simulink model "generic_src"  (Simulink 10.3)
settings: Solver=ode45  StartTime=0.0  StopTime=inf  RelTol=1e-3  EnableMultiTasking=on
undefined symbols (not defined in the file or in its folder): Area_Front, Area_Rear, ay_max_off, ay_max_on, ay_per_mu_max_off, ay_per_mu_max_on, Brake_ratio, brake_valve_ctrl_kP, cat1mode1_higher, cat1mode1_lower, cat1mode2_higher, cat1mode2_lower, cat1mode3_higher, cat1mode3_lower, cat2mode1_higher, cat2mode1_lower, cat2mode2_higher, cat2mode2_lower, cat2mode3_higher, cat2mode3_lower, delta_vel, diff_lock_fac, diff_lock_off, diff_lock_on, ESP_ctrl_kD, ESP_ctrl_kI, ESP_ctrl_kP, ESP_ctrl_restore_kI, ESP_min_throttle_fac, f_ax, f_slip, g, higherlimit_highvel, higherlimit_lowvel, highervel_fac, highervelocity_fac, InitialConditionForIntegrator, limit_acc, limit_selectlow, limit_starting, limit_vdiff, locktime_throttle, lowerlimit_highvel, lowerlimit_lowvel, lowervel_fac, lowervelocity_fac, min_throttle, MPS2KMPH, MSR_ctrl_kD, MSR_ctrl_kI, MSR_ctrl_kP, MSR_min_throttle_fac, PID_kP_sideslip, PID_kP_yawrate, RADpS2RpM, rBrake, RpM2RADpS, SH_SL_switch, sideslip_vel_corr, sidesplip_deviation_max ... (+35)
libraries: CarMaker4SL x136, simulink x55, simulink_extras x6
(part 6 of 9)

== system generic_src/CarMaker/IPG Vehicle/PowerTrain/PTControl Example/PTControl_In/CreateBus PTC_Cfg Gearbox10 ==
  In : Inport
  BusCreator : BusCreator  Inputs=38
  Demux : Demux  Outputs=38
      settings: DisplayOption=none
  Out : Outport  VectorParamsAs1DForOutWhenUnconnected=off
  wires:
  Demux/38 -> BusCreator/38  "PTC_Cfg Gearbox10 iBGear16"
  Demux/37 -> BusCreator/37  "PTC_Cfg Gearbox10 iBGear15"
  Demux/36 -> BusCreator/36  "PTC_Cfg Gearbox10 iBGear14"
  Demux/35 -> BusCreator/35  "PTC_Cfg Gearbox10 iBGear13"
  Demux/34 -> BusCreator/34  "PTC_Cfg Gearbox10 iBGear12"
  Demux/33 -> BusCreator/33  "PTC_Cfg Gearbox10 iBGear11"
  Demux/32 -> BusCreator/32  "PTC_Cfg Gearbox10 iBGear10"
  Demux/31 -> BusCreator/31  "PTC_Cfg Gearbox10 iBGear9"
  Demux/30 -> BusCreator/30  "PTC_Cfg Gearbox10 iBGear8"
  Demux/29 -> BusCreator/29  "PTC_Cfg Gearbox10 iBGear7"
  Demux/28 -> BusCreator/28  "PTC_Cfg Gearbox10 iBGear6"
  Demux/27 -> BusCreator/27  "PTC_Cfg Gearbox10 iBGear5"
  Demux/26 -> BusCreator/26  "PTC_Cfg Gearbox10 iBGear4"
  Demux/25 -> BusCreator/25  "PTC_Cfg Gearbox10 iBGear3"
  Demux/24 -> BusCreator/24  "PTC_Cfg Gearbox10 iBGear2"
  Demux/23 -> BusCreator/23  "PTC_Cfg Gearbox10 iBGear1"
  Demux/22 -> BusCreator/22  "PTC_Cfg Gearbox10 iBGear0"
  Demux/21 -> BusCreator/21  "PTC_Cfg Gearbox10 nBGears"
  Demux/20 -> BusCreator/20  "PTC_Cfg Gearbox10 iFGear16"
  Demux/19 -> BusCreator/19  "PTC_Cfg Gearbox10 iFGear15"
  Demux/18 -> BusCreator/18  "PTC_Cfg Gearbox10 iFGear14"
  Demux/17 -> BusCreator/17  "PTC_Cfg Gearbox10 iFGear13"
  Demux/16 -> BusCreator/16  "PTC_Cfg Gearbox10 iFGear12"
  Demux/15 -> BusCreator/15  "PTC_Cfg Gearbox10 iFGear11"
  Demux/14 -> BusCreator/14  "PTC_Cfg Gearbox10 iFGear10"
  Demux/13 -> BusCreator/13  "PTC_Cfg Gearbox10 iFGear9"
  Demux/12 -> BusCreator/12  "PTC_Cfg Gearbox10 iFGear8"
  Demux/11 -> BusCreator/11  "PTC_Cfg Gearbox10 iFGear7"
  Demux/10 -> BusCreator/10  "PTC_Cfg Gearbox10 iFGear6"
  Demux/9 -> BusCreator/9  "PTC_Cfg Gearbox10 iFGear5"
  Demux/8 -> BusCreator/8  "PTC_Cfg Gearbox10 iFGear4"
  Demux/7 -> BusCreator/7  "PTC_Cfg Gearbox10 iFGear3"
  Demux/6 -> BusCreator/6  "PTC_Cfg Gearbox10 iFGear2"
  Demux/5 -> BusCreator/5  "PTC_Cfg Gearbox10 iFGear1"
  Demux/4 -> BusCreator/4  "PTC_Cfg Gearbox10 iFGear0"
  Demux/3 -> BusCreator/3  "PTC_Cfg Gearbox10 nFGears"
  Demux/2 -> BusCreator/2  "PTC_Cfg Gearbox10 ClKind"
  Demux/1 -> BusCreator/1  "PTC_Cfg Gearbox10 GBKind"
  BusCreator/1 -> Out/1
  In/1 -> Demux/1

== system generic_src/CarMaker/IPG Vehicle/PowerTrain/PTControl Example/PTControl_In/CreateBus PTC_Cfg Gearbox11 ==
  In : Inport
  BusCreator : BusCreator  Inputs=38
  Demux : Demux  Outputs=38
      settings: DisplayOption=none
  Out : Outport  VectorParamsAs1DForOutWhenUnconnected=off
  wires:
  Demux/38 -> BusCreator/38  "PTC_Cfg Gearbox11 iBGear16"
  Demux/37 -> BusCreator/37  "PTC_Cfg Gearbox11 iBGear15"
  Demux/36 -> BusCreator/36  "PTC_Cfg Gearbox11 iBGear14"
  Demux/35 -> BusCreator/35  "PTC_Cfg Gearbox11 iBGear13"
  Demux/34 -> BusCreator/34  "PTC_Cfg Gearbox11 iBGear12"
  Demux/33 -> BusCreator/33  "PTC_Cfg Gearbox11 iBGear11"
  Demux/32 -> BusCreator/32  "PTC_Cfg Gearbox11 iBGear10"
  Demux/31 -> BusCreator/31  "PTC_Cfg Gearbox11 iBGear9"
  Demux/30 -> BusCreator/30  "PTC_Cfg Gearbox11 iBGear8"
  Demux/29 -> BusCreator/29  "PTC_Cfg Gearbox11 iBGear7"
  Demux/28 -> BusCreator/28  "PTC_Cfg Gearbox11 iBGear6"
  Demux/27 -> BusCreator/27  "PTC_Cfg Gearbox11 iBGear5"
  Demux/26 -> BusCreator/26  "PTC_Cfg Gearbox11 iBGear4"
  Demux/25 -> BusCreator/25  "PTC_Cfg Gearbox11 iBGear3"
  Demux/24 -> BusCreator/24  "PTC_Cfg Gearbox11 iBGear2"
  Demux/23 -> BusCreator/23  "PTC_Cfg Gearbox11 iBGear1"
  Demux/22 -> BusCreator/22  "PTC_Cfg Gearbox11 iBGear0"
  Demux/21 -> BusCreator/21  "PTC_Cfg Gearbox11 nBGears"
  Demux/20 -> BusCreator/20  "PTC_Cfg Gearbox11 iFGear16"
  Demux/19 -> BusCreator/19  "PTC_Cfg Gearbox11 iFGear15"
  Demux/18 -> BusCreator/18  "PTC_Cfg Gearbox11 iFGear14"
  Demux/17 -> BusCreator/17  "PTC_Cfg Gearbox11 iFGear13"
  Demux/16 -> BusCreator/16  "PTC_Cfg Gearbox11 iFGear12"
  Demux/15 -> BusCreator/15  "PTC_Cfg Gearbox11 iFGear11"
  Demux/14 -> BusCreator/14  "PTC_Cfg Gearbox11 iFGear10"
  Demux/13 -> BusCreator/13  "PTC_Cfg Gearbox11 iFGear9"
  Demux/12 -> BusCreator/12  "PTC_Cfg Gearbox11 iFGear8"
  Demux/11 -> BusCreator/11  "PTC_Cfg Gearbox11 iFGear7"
  Demux/10 -> BusCreator/10  "PTC_Cfg Gearbox11 iFGear6"
  Demux/9 -> BusCreator/9  "PTC_Cfg Gearbox11 iFGear5"
  Demux/8 -> BusCreator/8  "PTC_Cfg Gearbox11 iFGear4"
  Demux/7 -> BusCreator/7  "PTC_Cfg Gearbox11 iFGear3"
  Demux/6 -> BusCreator/6  "PTC_Cfg Gearbox11 iFGear2"
  Demux/5 -> BusCreator/5  "PTC_Cfg Gearbox11 iFGear1"
  Demux/4 -> BusCreator/4  "PTC_Cfg Gearbox11 iFGear0"
  Demux/3 -> BusCreator/3  "PTC_Cfg Gearbox11 nFGears"
  Demux/2 -> BusCreator/2  "PTC_Cfg Gearbox11 ClKind"
  Demux/1 -> BusCreator/1  "PTC_Cfg Gearbox11 GBKind"
  BusCreator/1 -> Out/1
  In/1 -> Demux/1

== system generic_src/CarMaker/IPG Vehicle/PowerTrain/PTControl Example/PTControl_In/CreateBus PTC_Cfg Gearbox2 ==
  In : Inport
  BusCreator : BusCreator  Inputs=38
  Demux : Demux  Outputs=38
      settings: DisplayOption=none
  Out : Outport  VectorParamsAs1DForOutWhenUnconnected=off
  wires:
  Demux/38 -> BusCreator/38  "PTC_Cfg Gearbox2 iBGear16"
  Demux/37 -> BusCreator/37  "PTC_Cfg Gearbox2 iBGear15"
  Demux/36 -> BusCreator/36  "PTC_Cfg Gearbox2 iBGear14"
  Demux/35 -> BusCreator/35  "PTC_Cfg Gearbox2 iBGear13"
  Demux/34 -> BusCreator/34  "PTC_Cfg Gearbox2 iBGear12"
  Demux/33 -> BusCreator/33  "PTC_Cfg Gearbox2 iBGear11"
  Demux/32 -> BusCreator/32  "PTC_Cfg Gearbox2 iBGear10"
  Demux/31 -> BusCreator/31  "PTC_Cfg Gearbox2 iBGear9"
  Demux/30 -> BusCreator/30  "PTC_Cfg Gearbox2 iBGear8"
  Demux/29 -> BusCreator/29  "PTC_Cfg Gearbox2 iBGear7"
  Demux/28 -> BusCreator/28  "PTC_Cfg Gearbox2 iBGear6"
  Demux/27 -> BusCreator/27  "PTC_Cfg Gearbox2 iBGear5"
  Demux/26 -> BusCreator/26  "PTC_Cfg Gearbox2 iBGear4"
  Demux/25 -> BusCreator/25  "PTC_Cfg Gearbox2 iBGear3"
  Demux/24 -> BusCreator/24  "PTC_Cfg Gearbox2 iBGear2"
  Demux/23 -> BusCreator/23  "PTC_Cfg Gearbox2 iBGear1"
  Demux/22 -> BusCreator/22  "PTC_Cfg Gearbox2 iBGear0"
  Demux/21 -> BusCreator/21  "PTC_Cfg Gearbox2 nBGears"
  Demux/20 -> BusCreator/20  "PTC_Cfg Gearbox2 iFGear16"
  Demux/19 -> BusCreator/19  "PTC_Cfg Gearbox2 iFGear15"
  Demux/18 -> BusCreator/18  "PTC_Cfg Gearbox2 iFGear14"
  Demux/17 -> BusCreator/17  "PTC_Cfg Gearbox2 iFGear13"
  Demux/16 -> BusCreator/16  "PTC_Cfg Gearbox2 iFGear12"
  Demux/15 -> BusCreator/15  "PTC_Cfg Gearbox2 iFGear11"
  Demux/14 -> BusCreator/14  "PTC_Cfg Gearbox2 iFGear10"
  Demux/13 -> BusCreator/13  "PTC_Cfg Gearbox2 iFGear9"
  Demux/12 -> BusCreator/12  "PTC_Cfg Gearbox2 iFGear8"
  Demux/11 -> BusCreator/11  "PTC_Cfg Gearbox2 iFGear7"
  Demux/10 -> BusCreator/10  "PTC_Cfg Gearbox2 iFGear6"
  Demux/9 -> BusCreator/9  "PTC_Cfg Gearbox2 iFGear5"
  Demux/8 -> BusCreator/8  "PTC_Cfg Gearbox2 iFGear4"
  Demux/7 -> BusCreator/7  "PTC_Cfg Gearbox2 iFGear3"
  Demux/6 -> BusCreator/6  "PTC_Cfg Gearbox2 iFGear2"
  Demux/5 -> BusCreator/5  "PTC_Cfg Gearbox2 iFGear1"
  Demux/4 -> BusCreator/4  "PTC_Cfg Gearbox2 iFGear0"
  Demux/3 -> BusCreator/3  "PTC_Cfg Gearbox2 nFGears"
  Demux/2 -> BusCreator/2  "PTC_Cfg Gearbox2 ClKind"
  Demux/1 -> BusCreator/1  "PTC_Cfg Gearbox2 GBKind"
  BusCreator/1 -> Out/1
  In/1 -> Demux/1

== system generic_src/CarMaker/IPG Vehicle/PowerTrain/PTControl Example/PTControl_In/CreateBus PTC_Cfg Gearbox3 ==
  In : Inport
  BusCreator : BusCreator  Inputs=38
  Demux : Demux  Outputs=38
      settings: DisplayOption=none
  Out : Outport  VectorParamsAs1DForOutWhenUnconnected=off
  wires:
  Demux/38 -> BusCreator/38  "PTC_Cfg Gearbox3 iBGear16"
  Demux/37 -> BusCreator/37  "PTC_Cfg Gearbox3 iBGear15"
  Demux/36 -> BusCreator/36  "PTC_Cfg Gearbox3 iBGear14"
  Demux/35 -> BusCreator/35  "PTC_Cfg Gearbox3 iBGear13"
  Demux/34 -> BusCreator/34  "PTC_Cfg Gearbox3 iBGear12"
  Demux/33 -> BusCreator/33  "PTC_Cfg Gearbox3 iBGear11"
  Demux/32 -> BusCreator/32  "PTC_Cfg Gearbox3 iBGear10"
  Demux/31 -> BusCreator/31  "PTC_Cfg Gearbox3 iBGear9"
  Demux/30 -> BusCreator/30  "PTC_Cfg Gearbox3 iBGear8"
  Demux/29 -> BusCreator/29  "PTC_Cfg Gearbox3 iBGear7"
  Demux/28 -> BusCreator/28  "PTC_Cfg Gearbox3 iBGear6"
  Demux/27 -> BusCreator/27  "PTC_Cfg Gearbox3 iBGear5"
  Demux/26 -> BusCreator/26  "PTC_Cfg Gearbox3 iBGear4"
  Demux/25 -> BusCreator/25  "PTC_Cfg Gearbox3 iBGear3"
  Demux/24 -> BusCreator/24  "PTC_Cfg Gearbox3 iBGear2"
  Demux/23 -> BusCreator/23  "PTC_Cfg Gearbox3 iBGear1"
  Demux/22 -> BusCreator/22  "PTC_Cfg Gearbox3 iBGear0"
  Demux/21 -> BusCreator/21  "PTC_Cfg Gearbox3 nBGears"
  Demux/20 -> BusCreator/20  "PTC_Cfg Gearbox3 iFGear16"
  Demux/19 -> BusCreator/19  "PTC_Cfg Gearbox3 iFGear15"
  Demux/18 -> BusCreator/18  "PTC_Cfg Gearbox3 iFGear14"
  Demux/17 -> BusCreator/17  "PTC_Cfg Gearbox3 iFGear13"
  Demux/16 -> BusCreator/16  "PTC_Cfg Gearbox3 iFGear12"
  Demux/15 -> BusCreator/15  "PTC_Cfg Gearbox3 iFGear11"
  Demux/14 -> BusCreator/14  "PTC_Cfg Gearbox3 iFGear10"
  Demux/13 -> BusCreator/13  "PTC_Cfg Gearbox3 iFGear9"
  Demux/12 -> BusCreator/12  "PTC_Cfg Gearbox3 iFGear8"
  Demux/11 -> BusCreator/11  "PTC_Cfg Gearbox3 iFGear7"
  Demux/10 -> BusCreator/10  "PTC_Cfg Gearbox3 iFGear6"
  Demux/9 -> BusCreator/9  "PTC_Cfg Gearbox3 iFGear5"
  Demux/8 -> BusCreator/8  "PTC_Cfg Gearbox3 iFGear4"
  Demux/7 -> BusCreator/7  "PTC_Cfg Gearbox3 iFGear3"
  Demux/6 -> BusCreator/6  "PTC_Cfg Gearbox3 iFGear2"
  Demux/5 -> BusCreator/5  "PTC_Cfg Gearbox3 iFGear1"
  Demux/4 -> BusCreator/4  "PTC_Cfg Gearbox3 iFGear0"
  Demux/3 -> BusCreator/3  "PTC_Cfg Gearbox3 nFGears"
  Demux/2 -> BusCreator/2  "PTC_Cfg Gearbox3 ClKind"
  Demux/1 -> BusCreator/1  "PTC_Cfg Gearbox3 GBKind"
  BusCreator/1 -> Out/1
  In/1 -> Demux/1

== system generic_src/CarMaker/IPG Vehicle/PowerTrain/PTControl Example/PTControl_In/CreateBus PTC_Cfg Gearbox4 ==
  In : Inport
  BusCreator : BusCreator  Inputs=38
  Demux : Demux  Outputs=38
      settings: DisplayOption=none
  Out : Outport  VectorParamsAs1DForOutWhenUnconnected=off
  wires:
  Demux/38 -> BusCreator/38  "PTC_Cfg Gearbox4 iBGear16"
  Demux/37 -> BusCreator/37  "PTC_Cfg Gearbox4 iBGear15"
  Demux/36 -> BusCreator/36  "PTC_Cfg Gearbox4 iBGear14"
  Demux/35 -> BusCreator/35  "PTC_Cfg Gearbox4 iBGear13"
  Demux/34 -> BusCreator/34  "PTC_Cfg Gearbox4 iBGear12"
  Demux/33 -> BusCreator/33  "PTC_Cfg Gearbox4 iBGear11"
  Demux/32 -> BusCreator/32  "PTC_Cfg Gearbox4 iBGear10"
  Demux/31 -> BusCreator/31  "PTC_Cfg Gearbox4 iBGear9"
  Demux/30 -> BusCreator/30  "PTC_Cfg Gearbox4 iBGear8"
  Demux/29 -> BusCreator/29  "PTC_Cfg Gearbox4 iBGear7"
  Demux/28 -> BusCreator/28  "PTC_Cfg Gearbox4 iBGear6"
  Demux/27 -> BusCreator/27  "PTC_Cfg Gearbox4 iBGear5"
  Demux/26 -> BusCreator/26  "PTC_Cfg Gearbox4 iBGear4"
  Demux/25 -> BusCreator/25  "PTC_Cfg Gearbox4 iBGear3"
  Demux/24 -> BusCreator/24  "PTC_Cfg Gearbox4 iBGear2"
  Demux/23 -> BusCreator/23  "PTC_Cfg Gearbox4 iBGear1"
  Demux/22 -> BusCreator/22  "PTC_Cfg Gearbox4 iBGear0"
  Demux/21 -> BusCreator/21  "PTC_Cfg Gearbox4 nBGears"
  Demux/20 -> BusCreator/20  "PTC_Cfg Gearbox4 iFGear16"
  Demux/19 -> BusCreator/19  "PTC_Cfg Gearbox4 iFGear15"
  Demux/18 -> BusCreator/18  "PTC_Cfg Gearbox4 iFGear14"
  Demux/17 -> BusCreator/17  "PTC_Cfg Gearbox4 iFGear13"
  Demux/16 -> BusCreator/16  "PTC_Cfg Gearbox4 iFGear12"
  Demux/15 -> BusCreator/15  "PTC_Cfg Gearbox4 iFGear11"
  Demux/14 -> BusCreator/14  "PTC_Cfg Gearbox4 iFGear10"
  Demux/13 -> BusCreator/13  "PTC_Cfg Gearbox4 iFGear9"
  Demux/12 -> BusCreator/12  "PTC_Cfg Gearbox4 iFGear8"
  Demux/11 -> BusCreator/11  "PTC_Cfg Gearbox4 iFGear7"
  Demux/10 -> BusCreator/10  "PTC_Cfg Gearbox4 iFGear6"
  Demux/9 -> BusCreator/9  "PTC_Cfg Gearbox4 iFGear5"
  Demux/8 -> BusCreator/8  "PTC_Cfg Gearbox4 iFGear4"
  Demux/7 -> BusCreator/7  "PTC_Cfg Gearbox4 iFGear3"
  Demux/6 -> BusCreator/6  "PTC_Cfg Gearbox4 iFGear2"
  Demux/5 -> BusCreator/5  "PTC_Cfg Gearbox4 iFGear1"
  Demux/4 -> BusCreator/4  "PTC_Cfg Gearbox4 iFGear0"
  Demux/3 -> BusCreator/3  "PTC_Cfg Gearbox4 nFGears"
  Demux/2 -> BusCreator/2  "PTC_Cfg Gearbox4 ClKind"
  Demux/1 -> BusCreator/1  "PTC_Cfg Gearbox4 GBKind"
  BusCreator/1 -> Out/1
  In/1 -> Demux/1

== system generic_src/CarMaker/IPG Vehicle/PowerTrain/PTControl Example/PTControl_In/CreateBus PTC_Cfg Gearbox5 ==
  In : Inport
  BusCreator : BusCreator  Inputs=38
  Demux : Demux  Outputs=38
      settings: DisplayOption=none
  Out : Outport  VectorParamsAs1DForOutWhenUnconnected=off
  wires:
  Demux/38 -> BusCreator/38  "PTC_Cfg Gearbox5 iBGear16"
  Demux/37 -> BusCreator/37  "PTC_Cfg Gearbox5 iBGear15"
  Demux/36 -> BusCreator/36  "PTC_Cfg Gearbox5 iBGear14"
  Demux/35 -> BusCreator/35  "PTC_Cfg Gearbox5 iBGear13"
  Demux/34 -> BusCreator/34  "PTC_Cfg Gearbox5 iBGear12"
  Demux/33 -> BusCreator/33  "PTC_Cfg Gearbox5 iBGear11"
  Demux/32 -> BusCreator/32  "PTC_Cfg Gearbox5 iBGear10"
  Demux/31 -> BusCreator/31  "PTC_Cfg Gearbox5 iBGear9"
  Demux/30 -> BusCreator/30  "PTC_Cfg Gearbox5 iBGear8"
  Demux/29 -> BusCreator/29  "PTC_Cfg Gearbox5 iBGear7"
  Demux/28 -> BusCreator/28  "PTC_Cfg Gearbox5 iBGear6"
  Demux/27 -> BusCreator/27  "PTC_Cfg Gearbox5 iBGear5"
  Demux/26 -> BusCreator/26  "PTC_Cfg Gearbox5 iBGear4"
  Demux/25 -> BusCreator/25  "PTC_Cfg Gearbox5 iBGear3"
  Demux/24 -> BusCreator/24  "PTC_Cfg Gearbox5 iBGear2"
  Demux/23 -> BusCreator/23  "PTC_Cfg Gearbox5 iBGear1"
  Demux/22 -> BusCreator/22  "PTC_Cfg Gearbox5 iBGear0"
  Demux/21 -> BusCreator/21  "PTC_Cfg Gearbox5 nBGears"
  Demux/20 -> BusCreator/20  "PTC_Cfg Gearbox5 iFGear16"
  Demux/19 -> BusCreator/19  "PTC_Cfg Gearbox5 iFGear15"
  Demux/18 -> BusCreator/18  "PTC_Cfg Gearbox5 iFGear14"
  Demux/17 -> BusCreator/17  "PTC_Cfg Gearbox5 iFGear13"
  Demux/16 -> BusCreator/16  "PTC_Cfg Gearbox5 iFGear12"
  Demux/15 -> BusCreator/15  "PTC_Cfg Gearbox5 iFGear11"
  Demux/14 -> BusCreator/14  "PTC_Cfg Gearbox5 iFGear10"
  Demux/13 -> BusCreator/13  "PTC_Cfg Gearbox5 iFGear9"
  Demux/12 -> BusCreator/12  "PTC_Cfg Gearbox5 iFGear8"
  Demux/11 -> BusCreator/11  "PTC_Cfg Gearbox5 iFGear7"
  Demux/10 -> BusCreator/10  "PTC_Cfg Gearbox5 iFGear6"
  Demux/9 -> BusCreator/9  "PTC_Cfg Gearbox5 iFGear5"
  Demux/8 -> BusCreator/8  "PTC_Cfg Gearbox5 iFGear4"
  Demux/7 -> BusCreator/7  "PTC_Cfg Gearbox5 iFGear3"
  Demux/6 -> BusCreator/6  "PTC_Cfg Gearbox5 iFGear2"
  Demux/5 -> BusCreator/5  "PTC_Cfg Gearbox5 iFGear1"
  Demux/4 -> BusCreator/4  "PTC_Cfg Gearbox5 iFGear0"
  Demux/3 -> BusCreator/3  "PTC_Cfg Gearbox5 nFGears"
  Demux/2 -> BusCreator/2  "PTC_Cfg Gearbox5 ClKind"
  Demux/1 -> BusCreator/1  "PTC_Cfg Gearbox5 GBKind"
  BusCreator/1 -> Out/1
  In/1 -> Demux/1

== system generic_src/CarMaker/IPG Vehicle/PowerTrain/PTControl Example/PTControl_In/CreateBus PTC_Cfg Gearbox6 ==
  In : Inport
  BusCreator : BusCreator  Inputs=38
  Demux : Demux  Outputs=38
      settings: DisplayOption=none
  Out : Outport  VectorParamsAs1DForOutWhenUnconnected=off
  wires:
  Demux/38 -> BusCreator/38  "PTC_Cfg Gearbox6 iBGear16"
  Demux/37 -> BusCreator/37  "PTC_Cfg Gearbox6 iBGear15"
  Demux/36 -> BusCreator/36  "PTC_Cfg Gearbox6 iBGear14"
  Demux/35 -> BusCreator/35  "PTC_Cfg Gearbox6 iBGear13"
  Demux/34 -> BusCreator/34  "PTC_Cfg Gearbox6 iBGear12"
  Demux/33 -> BusCreator/33  "PTC_Cfg Gearbox6 iBGear11"
  Demux/32 -> BusCreator/32  "PTC_Cfg Gearbox6 iBGear10"
  Demux/31 -> BusCreator/31  "PTC_Cfg Gearbox6 iBGear9"
  Demux/30 -> BusCreator/30  "PTC_Cfg Gearbox6 iBGear8"
  Demux/29 -> BusCreator/29  "PTC_Cfg Gearbox6 iBGear7"
  Demux/28 -> BusCreator/28  "PTC_Cfg Gearbox6 iBGear6"
  Demux/27 -> BusCreator/27  "PTC_Cfg Gearbox6 iBGear5"
  Demux/26 -> BusCreator/26  "PTC_Cfg Gearbox6 iBGear4"
  Demux/25 -> BusCreator/25  "PTC_Cfg Gearbox6 iBGear3"
  Demux/24 -> BusCreator/24  "PTC_Cfg Gearbox6 iBGear2"
  Demux/23 -> BusCreator/23  "PTC_Cfg Gearbox6 iBGear1"
  Demux/22 -> BusCreator/22  "PTC_Cfg Gearbox6 iBGear0"
  Demux/21 -> BusCreator/21  "PTC_Cfg Gearbox6 nBGears"
  Demux/20 -> BusCreator/20  "PTC_Cfg Gearbox6 iFGear16"
  Demux/19 -> BusCreator/19  "PTC_Cfg Gearbox6 iFGear15"
  Demux/18 -> BusCreator/18  "PTC_Cfg Gearbox6 iFGear14"
  Demux/17 -> BusCreator/17  "PTC_Cfg Gearbox6 iFGear13"
  Demux/16 -> BusCreator/16  "PTC_Cfg Gearbox6 iFGear12"
  Demux/15 -> BusCreator/15  "PTC_Cfg Gearbox6 iFGear11"
  Demux/14 -> BusCreator/14  "PTC_Cfg Gearbox6 iFGear10"
  Demux/13 -> BusCreator/13  "PTC_Cfg Gearbox6 iFGear9"
  Demux/12 -> BusCreator/12  "PTC_Cfg Gearbox6 iFGear8"
  Demux/11 -> BusCreator/11  "PTC_Cfg Gearbox6 iFGear7"
  Demux/10 -> BusCreator/10  "PTC_Cfg Gearbox6 iFGear6"
  Demux/9 -> BusCreator/9  "PTC_Cfg Gearbox6 iFGear5"
  Demux/8 -> BusCreator/8  "PTC_Cfg Gearbox6 iFGear4"
  Demux/7 -> BusCreator/7  "PTC_Cfg Gearbox6 iFGear3"
  Demux/6 -> BusCreator/6  "PTC_Cfg Gearbox6 iFGear2"
  Demux/5 -> BusCreator/5  "PTC_Cfg Gearbox6 iFGear1"
  Demux/4 -> BusCreator/4  "PTC_Cfg Gearbox6 iFGear0"
  Demux/3 -> BusCreator/3  "PTC_Cfg Gearbox6 nFGears"
  Demux/2 -> BusCreator/2  "PTC_Cfg Gearbox6 ClKind"
  Demux/1 -> BusCreator/1  "PTC_Cfg Gearbox6 GBKind"
  BusCreator/1 -> Out/1
  In/1 -> Demux/1

== system generic_src/CarMaker/IPG Vehicle/PowerTrain/PTControl Example/PTControl_In/CreateBus PTC_Cfg Gearbox7 ==
  In : Inport
  BusCreator : BusCreator  Inputs=38
  Demux : Demux  Outputs=38
      settings: DisplayOption=none
  Out : Outport  VectorParamsAs1DForOutWhenUnconnected=off
  wires:
  Demux/38 -> BusCreator/38  "PTC_Cfg Gearbox7 iBGear16"
  Demux/37 -> BusCreator/37  "PTC_Cfg Gearbox7 iBGear15"
  Demux/36 -> BusCreator/36  "PTC_Cfg Gearbox7 iBGear14"
  Demux/35 -> BusCreator/35  "PTC_Cfg Gearbox7 iBGear13"
  Demux/34 -> BusCreator/34  "PTC_Cfg Gearbox7 iBGear12"
  Demux/33 -> BusCreator/33  "PTC_Cfg Gearbox7 iBGear11"
  Demux/32 -> BusCreator/32  "PTC_Cfg Gearbox7 iBGear10"
  Demux/31 -> BusCreator/31  "PTC_Cfg Gearbox7 iBGear9"
  Demux/30 -> BusCreator/30  "PTC_Cfg Gearbox7 iBGear8"
  Demux/29 -> BusCreator/29  "PTC_Cfg Gearbox7 iBGear7"
  Demux/28 -> BusCreator/28  "PTC_Cfg Gearbox7 iBGear6"
  Demux/27 -> BusCreator/27  "PTC_Cfg Gearbox7 iBGear5"
  Demux/26 -> BusCreator/26  "PTC_Cfg Gearbox7 iBGear4"
  Demux/25 -> BusCreator/25  "PTC_Cfg Gearbox7 iBGear3"
  Demux/24 -> BusCreator/24  "PTC_Cfg Gearbox7 iBGear2"
  Demux/23 -> BusCreator/23  "PTC_Cfg Gearbox7 iBGear1"
  Demux/22 -> BusCreator/22  "PTC_Cfg Gearbox7 iBGear0"
  Demux/21 -> BusCreator/21  "PTC_Cfg Gearbox7 nBGears"
  Demux/20 -> BusCreator/20  "PTC_Cfg Gearbox7 iFGear16"
  Demux/19 -> BusCreator/19  "PTC_Cfg Gearbox7 iFGear15"
  Demux/18 -> BusCreator/18  "PTC_Cfg Gearbox7 iFGear14"
  Demux/17 -> BusCreator/17  "PTC_Cfg Gearbox7 iFGear13"
  Demux/16 -> BusCreator/16  "PTC_Cfg Gearbox7 iFGear12"
  Demux/15 -> BusCreator/15  "PTC_Cfg Gearbox7 iFGear11"
  Demux/14 -> BusCreator/14  "PTC_Cfg Gearbox7 iFGear10"
  Demux/13 -> BusCreator/13  "PTC_Cfg Gearbox7 iFGear9"
  Demux/12 -> BusCreator/12  "PTC_Cfg Gearbox7 iFGear8"
  Demux/11 -> BusCreator/11  "PTC_Cfg Gearbox7 iFGear7"
  Demux/10 -> BusCreator/10  "PTC_Cfg Gearbox7 iFGear6"
  Demux/9 -> BusCreator/9  "PTC_Cfg Gearbox7 iFGear5"
  Demux/8 -> BusCreator/8  "PTC_Cfg Gearbox7 iFGear4"
  Demux/7 -> BusCreator/7  "PTC_Cfg Gearbox7 iFGear3"
  Demux/6 -> BusCreator/6  "PTC_Cfg Gearbox7 iFGear2"
  Demux/5 -> BusCreator/5  "PTC_Cfg Gearbox7 iFGear1"
  Demux/4 -> BusCreator/4  "PTC_Cfg Gearbox7 iFGear0"
  Demux/3 -> BusCreator/3  "PTC_Cfg Gearbox7 nFGears"
  Demux/2 -> BusCreator/2  "PTC_Cfg Gearbox7 ClKind"
  Demux/1 -> BusCreator/1  "PTC_Cfg Gearbox7 GBKind"
  BusCreator/1 -> Out/1
  In/1 -> Demux/1

== system generic_src/CarMaker/IPG Vehicle/PowerTrain/PTControl Example/PTControl_In/CreateBus PTC_Cfg Gearbox8 ==
  In : Inport
  BusCreator : BusCreator  Inputs=38
  Demux : Demux  Outputs=38
      settings: DisplayOption=none
  Out : Outport  VectorParamsAs1DForOutWhenUnconnected=off
  wires:
  Demux/38 -> BusCreator/38  "PTC_Cfg Gearbox8 iBGear16"
  Demux/37 -> BusCreator/37  "PTC_Cfg Gearbox8 iBGear15"
  Demux/36 -> BusCreator/36  "PTC_Cfg Gearbox8 iBGear14"
  Demux/35 -> BusCreator/35  "PTC_Cfg Gearbox8 iBGear13"
  Demux/34 -> BusCreator/34  "PTC_Cfg Gearbox8 iBGear12"
  Demux/33 -> BusCreator/33  "PTC_Cfg Gearbox8 iBGear11"
  Demux/32 -> BusCreator/32  "PTC_Cfg Gearbox8 iBGear10"
  Demux/31 -> BusCreator/31  "PTC_Cfg Gearbox8 iBGear9"
  Demux/30 -> BusCreator/30  "PTC_Cfg Gearbox8 iBGear8"
  Demux/29 -> BusCreator/29  "PTC_Cfg Gearbox8 iBGear7"
  Demux/28 -> BusCreator/28  "PTC_Cfg Gearbox8 iBGear6"
  Demux/27 -> BusCreator/27  "PTC_Cfg Gearbox8 iBGear5"
  Demux/26 -> BusCreator/26  "PTC_Cfg Gearbox8 iBGear4"
  Demux/25 -> BusCreator/25  "PTC_Cfg Gearbox8 iBGear3"
  Demux/24 -> BusCreator/24  "PTC_Cfg Gearbox8 iBGear2"
  Demux/23 -> BusCreator/23  "PTC_Cfg Gearbox8 iBGear1"
  Demux/22 -> BusCreator/22  "PTC_Cfg Gearbox8 iBGear0"
  Demux/21 -> BusCreator/21  "PTC_Cfg Gearbox8 nBGears"
  Demux/20 -> BusCreator/20  "PTC_Cfg Gearbox8 iFGear16"
  Demux/19 -> BusCreator/19  "PTC_Cfg Gearbox8 iFGear15"
  Demux/18 -> BusCreator/18  "PTC_Cfg Gearbox8 iFGear14"
  Demux/17 -> BusCreator/17  "PTC_Cfg Gearbox8 iFGear13"
  Demux/16 -> BusCreator/16  "PTC_Cfg Gearbox8 iFGear12"
  Demux/15 -> BusCreator/15  "PTC_Cfg Gearbox8 iFGear11"
  Demux/14 -> BusCreator/14  "PTC_Cfg Gearbox8 iFGear10"
  Demux/13 -> BusCreator/13  "PTC_Cfg Gearbox8 iFGear9"
  Demux/12 -> BusCreator/12  "PTC_Cfg Gearbox8 iFGear8"
  Demux/11 -> BusCreator/11  "PTC_Cfg Gearbox8 iFGear7"
  Demux/10 -> BusCreator/10  "PTC_Cfg Gearbox8 iFGear6"
  Demux/9 -> BusCreator/9  "PTC_Cfg Gearbox8 iFGear5"
  Demux/8 -> BusCreator/8  "PTC_Cfg Gearbox8 iFGear4"
  Demux/7 -> BusCreator/7  "PTC_Cfg Gearbox8 iFGear3"
  Demux/6 -> BusCreator/6  "PTC_Cfg Gearbox8 iFGear2"
  Demux/5 -> BusCreator/5  "PTC_Cfg Gearbox8 iFGear1"
  Demux/4 -> BusCreator/4  "PTC_Cfg Gearbox8 iFGear0"
  Demux/3 -> BusCreator/3  "PTC_Cfg Gearbox8 nFGears"
  Demux/2 -> BusCreator/2  "PTC_Cfg Gearbox8 ClKind"
  Demux/1 -> BusCreator/1  "PTC_Cfg Gearbox8 GBKind"
  BusCreator/1 -> Out/1
  In/1 -> Demux/1

== system generic_src/CarMaker/IPG Vehicle/PowerTrain/PTControl Example/PTControl_In/CreateBus PTC_Cfg Gearbox9 ==
  In : Inport
  BusCreator : BusCreator  Inputs=38
  Demux : Demux  Outputs=38
      settings: DisplayOption=none
  Out : Outport  VectorParamsAs1DForOutWhenUnconnected=off
  wires:
  Demux/38 -> BusCreator/38  "PTC_Cfg Gearbox9 iBGear16"
  Demux/37 -> BusCreator/37  "PTC_Cfg Gearbox9 iBGear15"
  Demux/36 -> BusCreator/36  "PTC_Cfg Gearbox9 iBGear14"
  Demux/35 -> BusCreator/35  "PTC_Cfg Gearbox9 iBGear13"
  Demux/34 -> BusCreator/34  "PTC_Cfg Gearbox9 iBGear12"
  Demux/33 -> BusCreator/33  "PTC_Cfg Gearbox9 iBGear11"
  Demux/32 -> BusCreator/32  "PTC_Cfg Gearbox9 iBGear10"
  Demux/31 -> BusCreator/31  "PTC_Cfg Gearbox9 iBGear9"
  Demux/30 -> BusCreator/30  "PTC_Cfg Gearbox9 iBGear8"
  Demux/29 -> BusCreator/29  "PTC_Cfg Gearbox9 iBGear7"
  Demux/28 -> BusCreator/28  "PTC_Cfg Gearbox9 iBGear6"
  Demux/27 -> BusCreator/27  "PTC_Cfg Gearbox9 iBGear5"
  Demux/26 -> BusCreator/26  "PTC_Cfg Gearbox9 iBGear4"
  Demux/25 -> BusCreator/25  "PTC_Cfg Gearbox9 iBGear3"
  Demux/24 -> BusCreator/24  "PTC_Cfg Gearbox9 iBGear2"
  Demux/23 -> BusCreator/23  "PTC_Cfg Gearbox9 iBGear1"
  Demux/22 -> BusCreator/22  "PTC_Cfg Gearbox9 iBGear0"
  Demux/21 -> BusCreator/21  "PTC_Cfg Gearbox9 nBGears"
  Demux/20 -> BusCreator/20  "PTC_Cfg Gearbox9 iFGear16"
  Demux/19 -> BusCreator/19  "PTC_Cfg Gearbox9 iFGear15"
  Demux/18 -> BusCreator/18  "PTC_Cfg Gearbox9 iFGear14"
  Demux/17 -> BusCreator/17  "PTC_Cfg Gearbox9 iFGear13"
  Demux/16 -> BusCreator/16  "PTC_Cfg Gearbox9 iFGear12"
  Demux/15 -> BusCreator/15  "PTC_Cfg Gearbox9 iFGear11"
  Demux/14 -> BusCreator/14  "PTC_Cfg Gearbox9 iFGear10"
  Demux/13 -> BusCreator/13  "PTC_Cfg Gearbox9 iFGear9"
  Demux/12 -> BusCreator/12  "PTC_Cfg Gearbox9 iFGear8"
  Demux/11 -> BusCreator/11  "PTC_Cfg Gearbox9 iFGear7"
  Demux/10 -> BusCreator/10  "PTC_Cfg Gearbox9 iFGear6"
  Demux/9 -> BusCreator/9  "PTC_Cfg Gearbox9 iFGear5"
  Demux/8 -> BusCreator/8  "PTC_Cfg Gearbox9 iFGear4"
  Demux/7 -> BusCreator/7  "PTC_Cfg Gearbox9 iFGear3"
  Demux/6 -> BusCreator/6  "PTC_Cfg Gearbox9 iFGear2"
  Demux/5 -> BusCreator/5  "PTC_Cfg Gearbox9 iFGear1"
  Demux/4 -> BusCreator/4  "PTC_Cfg Gearbox9 iFGear0"
  Demux/3 -> BusCreator/3  "PTC_Cfg Gearbox9 nFGears"
  Demux/2 -> BusCreator/2  "PTC_Cfg Gearbox9 ClKind"
  Demux/1 -> BusCreator/1  "PTC_Cfg Gearbox9 GBKind"
  BusCreator/1 -> Out/1
  In/1 -> Demux/1

== system generic_src/CarMaker/IPG Vehicle/PowerTrain/PTControl Example/PTControl_In/CreateBus PTC_Cfg ISG1 ==
  In : Inport
  BusCreator : BusCreator  Inputs=9
  Demux : Demux  Outputs=9
      settings: DisplayOption=none
  Out : Outport  VectorParamsAs1DForOutWhenUnconnected=off
  wires:
  BusCreator/1 -> Out/1
  In/1 -> Demux/1
  Demux/5 -> BusCreator/5  "PTC_Cfg ISG rotv_Gen_max"
  Demux/4 -> BusCreator/4  "PTC_Cfg ISG rotv_Mot_max"
  Demux/3 -> BusCreator/3  "PTC_Cfg ISG Ratio"
  Demux/2 -> BusCreator/2  "PTC_Cfg ISG Level"
  Demux/1 -> BusCreator/1  "PTC_Cfg ISG CtrlMode"
  Demux/6 -> BusCreator/6  "PTC_Cfg ISG nPolePairs"
  Demux/7 -> BusCreator/7  "PTC_Cfg ISG L_d"
  Demux/8 -> BusCreator/8  "PTC_Cfg ISG _Lq"
  Demux/9 -> BusCreator/9  "PTC_Cfg ISG Psi_PM"

== system generic_src/CarMaker/IPG Vehicle/PowerTrain/PTControl Example/PTControl_In/CreateBus PTC_Cfg Misc ==
  In : Inport
  BusCreator : BusCreator  Inputs=14
  Demux : Demux  Outputs=14
      settings: DisplayOption=none
  Out : Outport  VectorParamsAs1DForOutWhenUnconnected=off
  wires:
  BusCreator/1 -> Out/1
  In/1 -> Demux/1
  Demux/4 -> BusCreator/4  "PTC_Cfg nClutch"
  Demux/11 -> BusCreator/11  "PTC_Cfg DriveSourcePos0"
  Demux/12 -> BusCreator/12  "PTC_Cfg DriveSourcePos1"
  Demux/14 -> BusCreator/14  "PTC_Cfg DriveSourcePos3"
  Demux/5 -> BusCreator/5  "PTC_Cfg nGearbox"
  Demux/2 -> BusCreator/2  "PTC_Cfg ClKind"
  Demux/10 -> BusCreator/10  "PTC_Cfg DL_iDiff_mean"
  Demux/9 -> BusCreator/9  "PTC_Cfg Aero_Frcx"
  Demux/1 -> BusCreator/1  "PTC_Cfg PTKind"
  Demux/8 -> BusCreator/8  "PTC_Cfg WheelRadius"
  Demux/13 -> BusCreator/13  "PTC_Cfg DriveSourcePos2"
  Demux/7 -> BusCreator/7  "PTC_Cfg Vehicle_nWheels"
  Demux/3 -> BusCreator/3  "PTC_Cfg nMotor"
  Demux/6 -> BusCreator/6  "PTC_Cfg nPlanetGear"

== system generic_src/CarMaker/IPG Vehicle/PowerTrain/PTControl Example/PTControl_In/CreateBus PTC_Cfg Motor1 ==
  In : Inport
  BusCreator : BusCreator  Inputs=108
  Demux : Demux  Outputs=108
      settings: DisplayOption=none
  Out : Outport  VectorParamsAs1DForOutWhenUnconnected=off
  wires:
  Demux/32 -> BusCreator/32  "PTC_Cfg Motor3 rotv_Gen_max"
  Demux/31 -> BusCreator/31  "PTC_Cfg Motor3 rotv_Mot_max"
  Demux/30 -> BusCreator/30  "PTC_Cfg Motor3 Ratio"
  Demux/29 -> BusCreator/29  "PTC_Cfg Motor3 Level"
  Demux/23 -> BusCreator/23  "PTC_Cfg Motor2 rotv_Gen_max"
  Demux/22 -> BusCreator/22  "PTC_Cfg Motor2 rotv_Mot_max"
  Demux/21 -> BusCreator/21  "PTC_Cfg Motor2 Ratio"
  Demux/14 -> BusCreator/14  "PTC_Cfg Motor1 rotv_Gen_max"
  Demux/13 -> BusCreator/13  "PTC_Cfg Motor1 rotv_Mot_max"
  Demux/12 -> BusCreator/12  "PTC_Cfg Motor1 Ratio"
  Demux/11 -> BusCreator/11  "PTC_Cfg Motor1 Level"
  BusCreator/1 -> Out/1
  In/1 -> Demux/1
  Demux/38 -> BusCreator/38  "PTC_Cfg Motor4 Level"
  Demux/39 -> BusCreator/39  "PTC_Cfg Motor4 Ratio"
  Demux/40 -> BusCreator/40  "PTC_Cfg Motor4 rotv_Mot_max"
  Demux/41 -> BusCreator/41  "PTC_Cfg Motor4 rotv_Gen_max"
  Demux/47 -> BusCreator/47  "PTC_Cfg Motor5 Level"
  Demux/48 -> BusCreator/48  "PTC_Cfg Motor5 Ratio"
  Demux/49 -> BusCreator/49  "PTC_Cfg Motor5 rotv_Mot_max"
  Demux/50 -> BusCreator/50  "PTC_Cfg Motor5 rotv_Gen_max"
  Demux/56 -> BusCreator/56  "PTC_Cfg Motor6 Level"
  Demux/57 -> BusCreator/57  "PTC_Cfg Motor6 Ratio"
  Demux/58 -> BusCreator/58  "PTC_Cfg Motor6 rotv_Mot_max"
  Demux/59 -> BusCreator/59  "PTC_Cfg Motor6 rotv_Gen_max"
  Demux/65 -> BusCreator/65  "PTC_Cfg Motor7 Level"
  Demux/66 -> BusCreator/66  "PTC_Cfg Motor7 Ratio"
  Demux/67 -> BusCreator/67  "PTC_Cfg Motor7 rotv_Mot_max"
  Demux/68 -> BusCreator/68  "PTC_Cfg Motor7 rotv_Gen_max"
  Demux/74 -> BusCreator/74  "PTC_Cfg Motor8 Level"
  Demux/75 -> BusCreator/75  "PTC_Cfg Motor8 Ratio"
  Demux/76 -> BusCreator/76  "PTC_Cfg Motor8 rotv_Mot_max"
  Demux/77 -> BusCreator/77  "PTC_Cfg Motor8 rotv_Gen_max"
  Demux/83 -> BusCreator/83  "PTC_Cfg Motor9 Level"
  Demux/84 -> BusCreator/84  "PTC_Cfg Motor9 Ratio"
  Demux/85 -> BusCreator/85  "PTC_Cfg Motor9 rotv_Mot_max"
  Demux/86 -> BusCreator/86  "PTC_Cfg Motor9 rotv_Gen_max"
  Demux/92 -> BusCreator/92  "PTC_Cfg Motor10 Level"
  Demux/93 -> BusCreator/93  "PTC_Cfg Motor10 Ratio"
  Demux/94 -> BusCreator/94  "PTC_Cfg Motor10 rotv_Mot_max"
  Demux/95 -> BusCreator/95  "PTC_Cfg Motor10 rotv_Gen_max"
  Demux/101 -> BusCreator/101  "PTC_Cfg Motor11 Level"
  Demux/102 -> BusCreator/102  "PTC_Cfg Motor11 Ratio"
  Demux/103 -> BusCreator/103  "PTC_Cfg Motor11 rotv_Mot_max"
  Demux/104 -> BusCreator/104  "PTC_Cfg Motor11 rotv_Gen_max"
  Demux/1 -> BusCreator/1  "PTC_Cfg Motor0 CtrlMode"
  Demux/5 -> BusCreator/5  "PTC_Cfg Motor0 rotv_Gen_max"
  Demux/4 -> BusCreator/4  "PTC_Cfg Motor0 rotv_Mot_max"
  Demux/3 -> BusCreator/3  "PTC_Cfg Motor0 Ratio"
  Demux/2 -> BusCreator/2  "PTC_Cfg Motor0 Level"
  Demux/6 -> BusCreator/6  "PTC_Cfg Motor0 nPolePairs"
  Demux/7 -> BusCreator/7  "PTC_Cfg Motor0 L_d"
  Demux/8 -> BusCreator/8  "PTC_Cfg Motor0 L_q"
  Demux/9 -> BusCreator/9  "PTC_Cfg Motor0 Psi_PM"
  Demux/10 -> BusCreator/10  "PTC_Cfg Motor1 CtrlMode"
  Demux/15 -> BusCreator/15  "PTC_Cfg Motor1 nPolePairs"
  Demux/16 -> BusCreator/16  "PTC_Cfg Motor1 L_d"
  Demux/17 -> BusCreator/17  "PTC_Cfg Motor1 L_q"
  Demux/18 -> BusCreator/18  "PTC_Cfg Motor1 Psi_PM"
  Demux/19 -> BusCreator/19  "PTC_Cfg Motor2 CtrlMode"
  Demux/20 -> BusCreator/20  "PTC_Cfg Motor2 Level"
  Demux/24 -> BusCreator/24  "PTC_Cfg Motor2 nPolePairs"
  Demux/25 -> BusCreator/25  "PTC_Cfg Motor2 L_d"
  Demux/26 -> BusCreator/26  "PTC_Cfg Motor2 L_q"
  Demux/27 -> BusCreator/27  "PTC_Cfg Motor2 Psi_PM"
  Demux/28 -> BusCreator/28  "PTC_Cfg Motor3 CtrlMode"
  Demux/33 -> BusCreator/33  "PTC_Cfg Motor3 nPolePairs"
  Demux/34 -> BusCreator/34  "PTC_Cfg Motor3 L_d"
  Demux/35 -> BusCreator/35  "PTC_Cfg Motor3 L_q"
  Demux/36 -> BusCreator/36  "PTC_Cfg Motor3 Psi_PM"
  Demux/37 -> BusCreator/37  "PTC_Cfg Motor4 CtrlMode"
  Demux/42 -> BusCreator/42  "PTC_Cfg Motor4 nPolePairs"
  Demux/43 -> BusCreator/43  "PTC_Cfg Motor4 L_d"
  Demux/44 -> BusCreator/44  "PTC_Cfg Motor4 L_q"
  Demux/45 -> BusCreator/45  "PTC_Cfg Motor4 Psi_PM"
  Demux/46 -> BusCreator/46  "PTC_Cfg Motor5 CtrlMode"
  Demux/51 -> BusCreator/51  "PTC_Cfg Motor5 nPolePairs"
  Demux/52 -> BusCreator/52  "PTC_Cfg Motor5 L_d"
  Demux/53 -> BusCreator/53  "PTC_Cfg Motor5 L_q"
  Demux/54 -> BusCreator/54  "PTC_Cfg Motor5 Psi_PM"
  Demux/55 -> BusCreator/55  "PTC_Cfg Motor6 CtrlMode"
  Demux/60 -> BusCreator/60  "PTC_Cfg Motor6 nPolePairs"
  Demux/61 -> BusCreator/61  "PTC_Cfg Motor6 L_d"
  Demux/62 -> BusCreator/62  "PTC_Cfg Motor6 L_q"
  Demux/63 -> BusCreator/63  "PTC_Cfg Motor6 Psi_PM"
  Demux/64 -> BusCreator/64  "PTC_Cfg Motor7 CtrlMode"
  Demux/69 -> BusCreator/69  "PTC_Cfg Motor7 nPolePairs"
  Demux/70 -> BusCreator/70  "PTC_Cfg Motor7 L_d"
  Demux/71 -> BusCreator/71  "PTC_Cfg Motor7 L_q"
  Demux/72 -> BusCreator/72  "PTC_Cfg Motor7 Psi_PM"
  Demux/73 -> BusCreator/73  "PTC_Cfg Motor8 CtrlMode"
  Demux/78 -> BusCreator/78  "PTC_Cfg Motor8 nPolePairs"
  Demux/79 -> BusCreator/79  "PTC_Cfg Motor8 L_d"
  Demux/80 -> BusCreator/80  "PTC_Cfg Motor8 L_q"
  Demux/81 -> BusCreator/81  "PTC_Cfg Motor8 Psi_PM"
  Demux/82 -> BusCreator/82  "PTC_Cfg Motor9 CtrlMode"
  Demux/87 -> BusCreator/87  "PTC_Cfg Motor9 nPolePairs"
  Demux/88 -> BusCreator/88  "PTC_Cfg Motor9 L_d"
  Demux/89 -> BusCreator/89  "PTC_Cfg Motor9 L_q"
  Demux/90 -> BusCreator/90  "PTC_Cfg Motor9 Psi_PM"
  Demux/91 -> BusCreator/91  "PTC_Cfg Motor10 CtrlMode"
  Demux/96 -> BusCreator/96  "PTC_Cfg Motor10 nPolePairs"
  Demux/97 -> BusCreator/97  "PTC_Cfg Motor10 L_d"
  Demux/98 -> BusCreator/98  "PTC_Cfg Motor10 L_q"
  Demux/99 -> BusCreator/99  "PTC_Cfg Motor10 Psi_PM"
  Demux/100 -> BusCreator/100  "PTC_Cfg Motor11 CtrlMode"
  Demux/105 -> BusCreator/105  "PTC_Cfg Motor11 nPolePairs"
  Demux/106 -> BusCreator/106  "PTC_Cfg Motor11 L_d"
  Demux/107 -> BusCreator/107  "PTC_Cfg Motor11 L_q"
  Demux/108 -> BusCreator/108  "PTC_Cfg Motor11 Psi_PM"

== system generic_src/CarMaker/IPG Vehicle/PowerTrain/PTControl Example/PTControl_In/CreateBus PTC_Cfg PlanetGear ==
  In : Inport
  BusCreator : BusCreator  Inputs=1
  Demux : Demux  Outputs=1
      settings: DisplayOption=none
  Out : Outport  VectorParamsAs1DForOutWhenUnconnected=off
  wires:
  Demux/1 -> BusCreator/1  "PTC_Cfg PlanetGear0 Ratio"
  BusCreator/1 -> Out/1
  In/1 -> Demux/1

== system generic_src/CarMaker/IPG Vehicle/Brake/HydBrakeCU Example/ESP Controller/ESP General System/ABS ==
  note: ABS disabled when slower than v_min
  ABS Signal Bus : Inport
  Ideal_In : Inport  Port=2
  Vehicle Params : Inport  Port=3
  User_In : Inport  Port=4
  ABS ECU : Subsystem
  Bus Creator : BusCreator  Inputs=8
  Bus Creator2 : BusCreator  Inputs=2
  Bus Creator3 : BusCreator  Inputs=2
  Bus Selector3 : BusSelector  OutputSignals=ax [m/s^2],WheelSpeeds
  Bus Selector1 : BusSelector  OutputSignals=TireRadius
  Bus Selector2 : BusSelector  OutputSignals=Param_RadiusRR,Param_RadiusRL,Param_RadiusFR,Param_RadiusFL
  Bus Selector4 : BusSelector  OutputSignals=WheelSpd_RR,WheelSpd_RL,WheelSpd_FR,WheelSpd_FL
  helpsignals estimator : Subsystem
  ABS On : Outport  VectorParamsAs1DForOutWhenUnconnected=off
  Pilot Valves : Outport  Port=2  VectorParamsAs1DForOutWhenUnconnected=off
  Suction Valves : Outport  Port=3  VectorParamsAs1DForOutWhenUnconnected=off
  Brake Valves : Outport  Port=4  VectorParamsAs1DForOutWhenUnconnected=off
  Pump Ctrl : Outport  Port=5  VectorParamsAs1DForOutWhenUnconnected=off
  wires:
  helpsignals estimator/1(vref) -> ABS ECU/1(vref)
  helpsignals estimator/2(LongSlip_FL) -> ABS ECU/2(LongSlip_FL)
  helpsignals estimator/3(LongSlip_FR) -> ABS ECU/3(LongSlip_FR)
  helpsignals estimator/4(LongSlip_RL) -> ABS ECU/4(LongSlip_RL)
  ABS ECU/1(Brake Pump Ctrl) -> Pump Ctrl/1
  helpsignals estimator/5(LongSlip_RR) -> ABS ECU/5(LongSlip_RR)
  ABS ECU/10(ABS On) -> ABS On/1
  Bus Selector3/2 -> Bus Selector4/1, helpsignals estimator/4(WheelSpeeds)  "<WheelSpeeds>"
  Bus Creator/1 -> Brake Valves/1
  ABS ECU/2(Brake Valve_In_FL) -> Bus Creator/1  "Valve_In_FL"
  ABS ECU/3(Brake Valve_In_FR) -> Bus Creator/2  "Valve_In_FR"
  ABS ECU/4(Brake Valve_In_RL) -> Bus Creator/3  "Valve_In_RL"
  ABS ECU/5(Brake Valve_In_RR) -> Bus Creator/4  "Valve_In_RR"
  ABS ECU/6(Brake Valve_Out_FL) -> Bus Creator/5  "Valve_Out_FL"
  ABS ECU/7(Brake Valve_Out_FR) -> Bus Creator/6  "Valve_Out_FR"
  ABS ECU/8(Brake Valve_Out_RL) -> Bus Creator/7  "Valve_Out_RL"
  ABS ECU/9(Brake Valve_Out_RR) -> Bus Creator/8  "Valve_Out_RR"
  ABS ECU/11(Valve_PV_0) -> Bus Creator2/1  "Valve_PV_0"
  ABS ECU/12(Valve_PV_1) -> Bus Creator2/2  "Valve_PV_1"
  ABS ECU/13(Valve_SV_0) -> Bus Creator3/1  "Valve_SV_0"
  ABS ECU/14(Valve_SV_1) -> Bus Creator3/2  "Valve_SV_1"
  Bus Creator2/1 -> Pilot Valves/1
  Bus Creator3/1 -> Suction Valves/1
  User_In/1 -> helpsignals estimator/1(User_In)
  Bus Selector2/4 -> ABS ECU/10(radius_FL)  "<Param_RadiusFL>"
  Vehicle Params/1 -> Bus Selector1/1
  Bus Selector2/3 -> ABS ECU/11(radius_FR)  "<Param_RadiusFR>"
  Bus Selector2/2 -> ABS ECU/12(radius_RL)  "<Param_RadiusRL>"
  Bus Selector2/1 -> ABS ECU/13(radius_RR)  "<Param_RadiusRR>"
  Bus Selector1/1 -> Bus Selector2/1, helpsignals estimator/5(TireRadius)  "<TireRadius>"
  ABS Signal Bus/1 -> Bus Selector3/1
  Bus Selector3/1 -> helpsignals estimator/3(ax)  "<ax [m/s^2]>"
  Ideal_In/1 -> helpsignals estimator/2(Ideal_In)
  Bus Selector4/4 -> ABS ECU/6(Speed_FL)  "<WheelSpd_FL>"
  Bus Selector4/3 -> ABS ECU/7(Speed_FR)  "<WheelSpd_FR>"
  Bus Selector4/2 -> ABS ECU/8(Speed_RL)  "<WheelSpd_RL>"
  Bus Selector4/1 -> ABS ECU/9(Speed_RR)  "<WheelSpd_RR>"

== system generic_src/CarMaker/IPG Vehicle/Brake/HydBrakeCU Example/ESP Controller/ESP General System/ASR ==
  ASR Signal Bus : Inport
  Ideal_In : Inport  Port=2
  Vehicle Params : Inport  Port=3
  User_In : Inport  Port=4
  BMR ECU : Subsystem
  Bus Creator : BusCreator  Inputs=4
  Bus Creator3 : BusCreator  Inputs=3
  Bus Selector3 : BusSelector  OutputSignals=Throttle Valve Position,WheelSpeeds
  Bus Selector : BusSelector  OutputSignals=WheelSpd_FL,WheelSpd_FR,WheelSpd_RL,WheelSpd_RR
  Bus Selector1 : BusSelector  OutputSignals=TireRadius
  Bus Selector2 : BusSelector  OutputSignals=Param_RadiusFL,Param_RadiusFR,Param_RadiusRL,Param_RadiusRR
  Constant4 : Constant  Value=MPS2KMPH
  Logical Operator2 : Logic  Operator=OR  AllPortsSameDT=off
  MSR ECU : Subsystem
  Mux1 : Mux
  Product : Product  RndMeth=Zero
  Product1 : Product  RndMeth=Zero
  ASR On : Outport  VectorParamsAs1DForOutWhenUnconnected=off
  Pilot Valves : Outport  Port=2  VectorParamsAs1DForOutWhenUnconnected=off
  Suction Valves : Outport  Port=3  VectorParamsAs1DForOutWhenUnconnected=off
  Brake Valves : Outport  Port=4  VectorParamsAs1DForOutWhenUnconnected=off
  Pump Ctrl : Outport  Port=5  VectorParamsAs1DForOutWhenUnconnected=off
  Gas_out : Outport  Port=6  VectorParamsAs1DForOutWhenUnconnected=off
  Diff_Torque : Outport  Port=7  VectorParamsAs1DForOutWhenUnconnected=off
  wires:
  Product/1 -> Product1/1
  Bus Selector/1 -> Bus Creator/1  "<WheelSpd_FL>"
  Bus Selector/2 -> Bus Creator/2  "<WheelSpd_FR>"
  Bus Selector/3 -> Bus Creator/3  "<WheelSpd_RL>"
  Bus Selector/4 -> Bus Creator/4  "<WheelSpd_RR>"
  Bus Selector2/1 -> Mux1/1  "<Param_RadiusFL>"
  MSR ECU/2(MSR On) -> Bus Creator3/1, Logical Operator2/1  "MSR On"
  BMR ECU/1(BMR On) -> Logical Operator2/2, Bus Creator3/3  "BMR On"
  BMR ECU/2(Brake Valves) -> Brake Valves/1
  Product1/1 -> BMR ECU/2(WheelVelocity [kmph]), MSR ECU/2(WheelVelocity [kmph])
  Bus Creator/1 -> Product/1
  Mux1/1 -> Product/2
  MSR ECU/1(Gas_out) -> Gas_out/1
  Bus Creator3/1 -> ASR On/1
  Logical Operator2/1 -> Bus Creator3/2  "ASR On"
  BMR ECU/3(Pilot Valves) -> Pilot Valves/1
  BMR ECU/4(Suctions Valves) -> Suction Valves/1
  BMR ECU/5(Pump Ctrl) -> Pump Ctrl/1
  User_In/1 -> MSR ECU/3(User_In), BMR ECU/3(User_In)
  BMR ECU/6(Diff_Torque) -> Diff_Torque/1  "Diff_Torque"
  Vehicle Params/1 -> Bus Selector1/1
  Bus Selector2/2 -> Mux1/2  "<Param_RadiusFR>"
  Bus Selector2/3 -> Mux1/3  "<Param_RadiusRL>"
  Bus Selector2/4 -> Mux1/4  "<Param_RadiusRR>"
  Bus Selector1/1 -> Bus Selector2/1  "<TireRadius>"
  ASR Signal Bus/1 -> Bus Selector3/1
  Bus Selector3/1 -> BMR ECU/1(Throttle), MSR ECU/1(Throttle Position)  "<Throttle Valve Position>"
  Ideal_In/1 -> MSR ECU/4(Ideal_In), BMR ECU/4(Ideal_In)
  Constant4/1 -> Product1/2
  Bus Selector3/2 -> Bus Selector/1  "<WheelSpeeds>"

== system generic_src/CarMaker/IPG Vehicle/Brake/HydBrakeCU Example/ESP Controller/ESP General System/ESP ==
  ESP Signal Bus : Inport
  Ideal_In : Inport  Port=2
  Vehicle Params : Inport  Port=3
  User_In : Inport  Port=4
  Actuator Brake : Subsystem
  Bus Creator : BusCreator  Inputs=8
  Bus Creator1 : BusCreator  Inputs=2
  Bus Creator2 : BusCreator  Inputs=2
  Bus Selector1 : BusSelector  OutputSignals=ax [m/s^2],Throttle Valve Position,Yaw Rate,Steer Angle,ay [m/s^2],Wheel Cylinder Pressure
  ECU : Subsystem
  helpsignals estimator : Subsystem
  ESP On : Outport  VectorParamsAs1DForOutWhenUnconnected=off
  Pilot Valves : Outport  Port=2  VectorParamsAs1DForOutWhenUnconnected=off
  Suction Valves : Outport  Port=3  VectorParamsAs1DForOutWhenUnconnected=off
  Brake Valves : Outport  Port=4  VectorParamsAs1DForOutWhenUnconnected=off
  Pump Ctrl : Outport  Port=5  VectorParamsAs1DForOutWhenUnconnected=off
  Gas_Out : Outport  Port=6  VectorParamsAs1DForOutWhenUnconnected=off
  wires:
  ECU/2(FL_active) -> Actuator Brake/1(FL_active)
  ECU/3(FL_Trq_target) -> Actuator Brake/2(FL_Trq_target)
  ECU/4(FR_active) -> Actuator Brake/3(FR_active)
  ECU/5(FR_Trq_target) -> Actuator Brake/4(FR_Trq_target)
  ECU/6(RL_active) -> Actuator Brake/5(RL_active)
  ECU/7(RL_Trq_target) -> Actuator Brake/6(RL_Trq_target)
  ECU/8(RR_active) -> Actuator Brake/7(RR_active)
  ECU/9(RR_Trq_target) -> Actuator Brake/8(RR_Trq_target)
  helpsignals estimator/1(SideslipAngle) -> ECU/5(Sideslip)
  helpsignals estimator/2(mu) -> ECU/6(mu)
  Bus Selector1/4 -> ECU/4(Steer Angle), helpsignals estimator/1(Steer Angle)  "<Steer Angle>"
  Actuator Brake/1(Valve_In_FL) -> Bus Creator/1  "Valve_In_FL"
  Actuator Brake/2(Valve_In_FR) -> Bus Creator/2  "Valve_In_FR"
  Bus Selector1/1 -> ECU/1(ax)  "<ax [m/s^2]>"
  Actuator Brake/3(Valve_In_RL) -> Bus Creator/3  "Valve_In_RL"
  Actuator Brake/4(Valve_In_RR) -> Bus Creator/4  "Valve_In_RR"
  Bus Selector1/2 -> ECU/2(Throttle Position)  "<Throttle Valve Position>"
  Actuator Brake/5(Valve_Out_FL) -> Bus Creator/5  "Valve_Out_FL"
  Actuator Brake/6(Valve_Out_FR) -> Bus Creator/6  "Valve_Out_FR"
  Bus Selector1/3 -> ECU/3(Yaw Rate)  "<Yaw Rate>"
  Actuator Brake/7(Valve_Out_RL) -> Bus Creator/7  "Valve_Out_RL"
  Actuator Brake/8(Valve_Out_RR) -> Bus Creator/8  "Valve_Out_RR"
  Actuator Brake/9(Valve_PV_0) -> Bus Creator2/1  "Valve_PV_0"
  Actuator Brake/10(Valve_PV_1) -> Bus Creator2/2  "Valve_PV_1"
  Actuator Brake/11(Valve_SV_0) -> Bus Creator1/1  "Valve_SV_0"
  Actuator Brake/12(Valve_SV_1) -> Bus Creator1/2  "Valve_SV_1"
  Actuator Brake/13(PumpCtrl) -> Pump Ctrl/1  "PumpCtrl"
  Actuator Brake/14(ESP_On) -> ESP On/1  "ESP_On"
  ECU/1(Gas_out) -> Gas_Out/1
  Bus Creator/1 -> Brake Valves/1
  Bus Creator2/1 -> Pilot Valves/1
  Bus Creator1/1 -> Suction Valves/1
  User_In/1 -> ECU/10(User_In), helpsignals estimator/4(User_In)
  Ideal_In/1 -> ECU/8(Ideal_In), helpsignals estimator/2(Ideal_In)
  Bus Selector1/6 -> Actuator Brake/9(Wheel Cylinder Pressure)  "<Wheel Cylinder Pressure>"
  Vehicle Params/1 -> ECU/9(Vehicle Params), helpsignals estimator/3(Vehicle Params)
  ESP Signal Bus/1 -> Bus Selector1/1
  Bus Selector1/5 -> ECU/7(ay)  "<ay [m/s^2]>"

== system generic_src/CarMaker/IPG Vehicle/Brake/HydBrakeCU Example/ESP Controller/ESP General System/HSA ==
  HSA Signal Bus : Inport
  Ideal_In : Inport  Port=2
  Bus Selector2 : BusSelector  OutputSignals=Engine crankshaft output torque [Nm]
  Bus Selector1 : BusSelector  OutputSignals=Ideal_Pitch,Ideal_Velocity.Ideal_Velocity_x
  Data Type Conversion : DataTypeConversion
  Gain : Gain  Gain=-1
  Logical Operator : Logic  Inputs=3  AllPortsSameDT=off  OutDataTypeStr=boolean
  Relay : Relay  OnSwitchValue=threshold_carpitch_on  OffSwitchValue=threshold_carpitch_off
  Relay1 : Relay  OnSwitchValue=threshold_velocity_on  OffSwitchValue=threshold_velocity_off  OnOutputValue=0  OffOutputValue=1
  Relay2 : Relay  OnSwitchValue=threshold_eng_trq_on  OffSwitchValue=threshold_eng_trq_off  OnOutputValue=0  OffOutputValue=1
  HSA On : Outport  VectorParamsAs1DForOutWhenUnconnected=off
  BrakePark_Out : Outport  Port=2  VectorParamsAs1DForOutWhenUnconnected=off
  wires:
  Ideal_In/1 -> Bus Selector1/1
  Bus Selector1/1 -> Gain/1  "<Ideal_Pitch>"
  Gain/1 -> Relay/1
  Bus Selector1/2 -> Relay1/1  "<Ideal_Velocity_x>"
  Relay2/1 -> Logical Operator/1
  Relay1/1 -> Logical Operator/3
  Relay/1 -> Logical Operator/2
  Logical Operator/1 -> Data Type Conversion/1
  Data Type Conversion/1 -> HSA On/1, BrakePark_Out/1
  HSA Signal Bus/1 -> Bus Selector2/1
  Bus Selector2/1 -> Relay2/1  "<Engine crankshaft output torque [Nm]>"

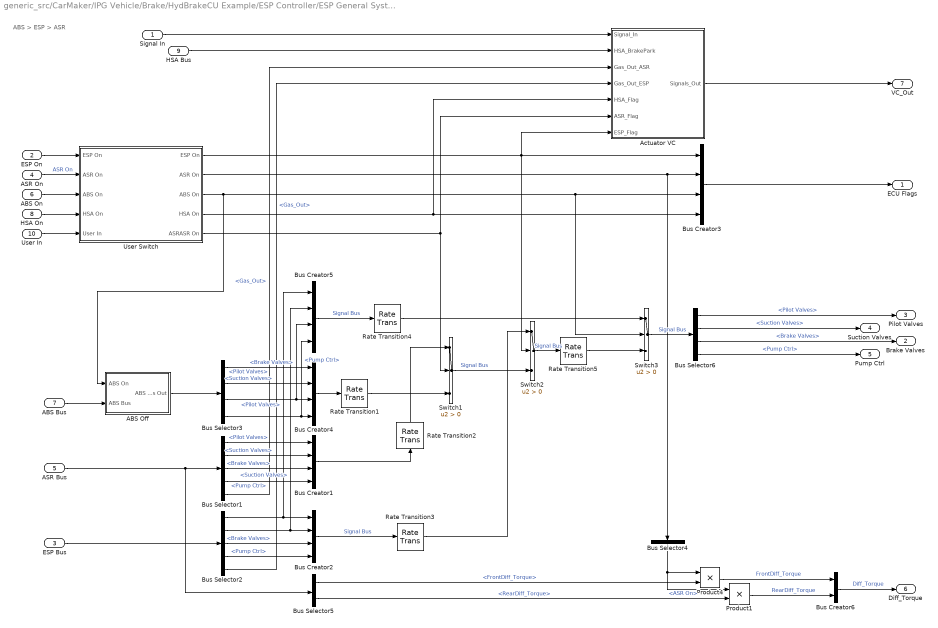
== system generic_src/CarMaker/IPG Vehicle/Brake/HydBrakeCU Example/ESP Controller/ESP General System/Master Controller ==
  note: ABS > ESP > ASR
  Signal In : Inport
  ESP On : Inport  Port=2
  ESP Bus : Inport  Port=3
  ASR On : Inport  Port=4
  ASR Bus : Inport  Port=5
  ABS On : Inport  Port=6
  ABS Bus : Inport  Port=7
  HSA On : Inport  Port=8
  HSA Bus : Inport  Port=9
  User In : Inport  Port=10
  ABS Off : Subsystem
  Actuator VC : Subsystem
  Bus Creator{1..5} (5 alike) : BusCreator  Inputs=4
  Bus Creator6 : BusCreator  Inputs=2
  Bus Selector1 : BusSelector  OutputSignals=Pilot Valves,Suction Valves,Brake Valves,Pump Ctrl,Gas_Out
  Bus Selector2 : BusSelector  OutputSignals=Pilot Valves,Suction Valves,Brake Valves,Pump Ctrl,Gas_Out
  Bus Selector3 : BusSelector  OutputSignals=Pilot Valves,Suction Valves,Brake Valves,Pump Ctrl
  Bus Selector4 : BusSelector  OutputSignals=ASR On
  Bus Selector5 : BusSelector  OutputSignals=Diff_Torque.FrontDiff_Torque,Diff_Torque.RearDiff_Torque
  Bus Selector6 : BusSelector  OutputSignals=Pilot Valves,Suction Valves,Brake Valves,Pump Ctrl
  Product1 : Product  RndMeth=Zero
  Product4 : Product  RndMeth=Zero
  Rate Transition{1..5} (5 alike) : RateTransition
  Switch1 : Switch  Criteria=u2 > Threshold
  Switch2 : Switch  Criteria=u2 > Threshold
  Switch3 : Switch  Criteria=u2 > Threshold
  User Switch : Subsystem
  ECU Flags : Outport  VectorParamsAs1DForOutWhenUnconnected=off
  Brake Valves : Outport  Port=2  VectorParamsAs1DForOutWhenUnconnected=off
  Pilot Valves : Outport  Port=3  VectorParamsAs1DForOutWhenUnconnected=off
  Suction Valves : Outport  Port=4  VectorParamsAs1DForOutWhenUnconnected=off
  Pump Ctrl : Outport  Port=5  VectorParamsAs1DForOutWhenUnconnected=off
  Diff_Torque : Outport  Port=6  VectorParamsAs1DForOutWhenUnconnected=off
  VC_Out : Outport  Port=7  VectorParamsAs1DForOutWhenUnconnected=off
  wires:
  Bus Creator3/1 -> ECU Flags/1
  Actuator VC/1(Signals_Out) -> VC_Out/1
  Signal In/1 -> Actuator VC/1(Signal_In)
  ESP Bus/1 -> Bus Selector2/1
  Bus Selector2/1 -> Bus Creator5/1, Bus Creator2/1  "<Pilot Valves>"
  Bus Selector2/2 -> Bus Creator5/2, Bus Creator2/2  "<Suction Valves>"
  Bus Selector2/3 -> Bus Creator2/3  "<Brake Valves>"
  Bus Selector2/4 -> Bus Creator2/4  "<Pump Ctrl>"
  Bus Selector6/1 -> Pilot Valves/1  "<Pilot Valves>"
  Bus Selector6/2 -> Suction Valves/1  "<Suction Valves>"
  Bus Selector6/3 -> Brake Valves/1  "<Brake Valves>"
  Bus Selector6/4 -> Pump Ctrl/1  "<Pump Ctrl>"
  Bus Selector3/3 -> Bus Creator5/3, Bus Creator4/3  "<Brake Valves>"
  Bus Selector3/4 -> Bus Creator5/4, Bus Creator4/4  "<Pump Ctrl>"
  ABS Bus/1 -> ABS Off/2(ABS Bus)
  Bus Selector3/1 -> Bus Creator4/1  "<Pilot Valves>"
  Bus Selector3/2 -> Bus Creator4/2  "<Suction Valves>"
  Switch1/1 -> Switch2/3  "Signal Bus"
  Bus Creator2/1 -> Rate Transition3/1  "Signal Bus"
  ASR Bus/1 -> Bus Selector5/1, Bus Selector1/1
  Bus Selector1/1 -> Bus Creator1/1  "<Pilot Valves>"
  Bus Selector1/2 -> Bus Creator1/2  "<Suction Valves>"
  Bus Selector1/3 -> Bus Creator1/3  "<Brake Valves>"
  Bus Selector1/4 -> Bus Creator1/4  "<Pump Ctrl>"
  Switch2/1 -> Rate Transition5/1  "Signal Bus"
  Bus Creator5/1 -> Rate Transition4/1  "Signal Bus"
  Bus Creator1/1 -> Rate Transition2/1
  Bus Creator4/1 -> Rate Transition1/1
  Rate Transition2/1 -> Switch1/1
  Rate Transition1/1 -> Switch1/3
  Switch3/1 -> Bus Selector6/1  "Signal Bus"
  Bus Selector1/5 -> Actuator VC/3(Gas_Out_ASR)  "<Gas_Out>"
  Bus Selector2/5 -> Actuator VC/4(Gas_Out_ESP)  "<Gas_Out>"
  User Switch/3("ABS On ") -> ABS Off/1(ABS On), Bus Creator3/3, Switch3/2
  User Switch/5(ASRASR On) -> Actuator VC/6(ASR_Flag), Switch1/2
  User Switch/1("ESP On ") -> Actuator VC/7(ESP_Flag), Bus Creator3/1, Switch2/2
  ESP On/1 -> User Switch/1(ESP On)
  ASR On/1 -> User Switch/2(ASR On)  "ASR On"
  ABS On/1 -> User Switch/3(ABS On)
  User In/1 -> User Switch/5(User In)
  User Switch/2("ASR On ") -> Bus Creator3/2, Bus Selector4/1
  HSA Bus/1 -> Actuator VC/2(HSA_BrakePark)
  HSA On/1 -> User Switch/4(HSA On)
  User Switch/4("HSA On ") -> Bus Creator3/4, Actuator VC/5(HSA_Flag)
  Bus Selector5/1 -> Product4/2  "<FrontDiff_Torque>"
  Bus Selector5/2 -> Product1/2  "<RearDiff_Torque>"
  Product4/1 -> Bus Creator6/1  "FrontDiff_Torque"
  Product1/1 -> Bus Creator6/2  "RearDiff_Torque"
  Bus Creator6/1 -> Diff_Torque/1  "Diff_Torque"
  Bus Selector4/1 -> Product1/1, Product4/1  "<ASR On>"
  ABS Off/1(ABS Bus Out) -> Bus Selector3/1
  Rate Transition3/1 -> Switch2/1
  Rate Transition4/1 -> Switch3/1
  Rate Transition5/1 -> Switch3/3
